simulink model "single_motor_fix"  (R2025b)
settings: Solver=VariableStepAuto  StartTime=0.0  StopTime=10.0  RelTol=1e-3
values from neighbouring files (symbols this model uses):
  Dm = 1e-3    (= 0.001)    [motor_param.m]
  Jm = 0.1e-3    (= 0.0001)    [motor_param.m]
  Ld = 0.01    [motor_param.m]
  Lq = 0.02    [motor_param.m]
  p = 2    [motor_param.m]
  Phi = 0.1    [motor_param.m]
  Rs = 0.38    [motor_param.m]
libraries: fl_lib x20, nesl_utility x20, ee_lib x6, eeTransforms x4, simulink x2
(part 1 of 2)
settings Model: Creator=ZhiyongXu  LastModifiedBy=ZhiyongXu

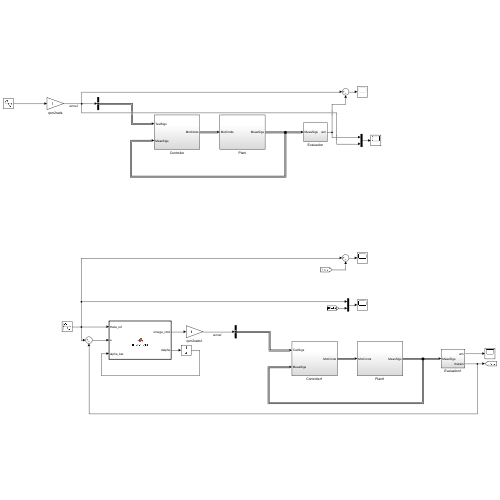
[thumbnail: Simulink's stored preview of the top-level diagram]
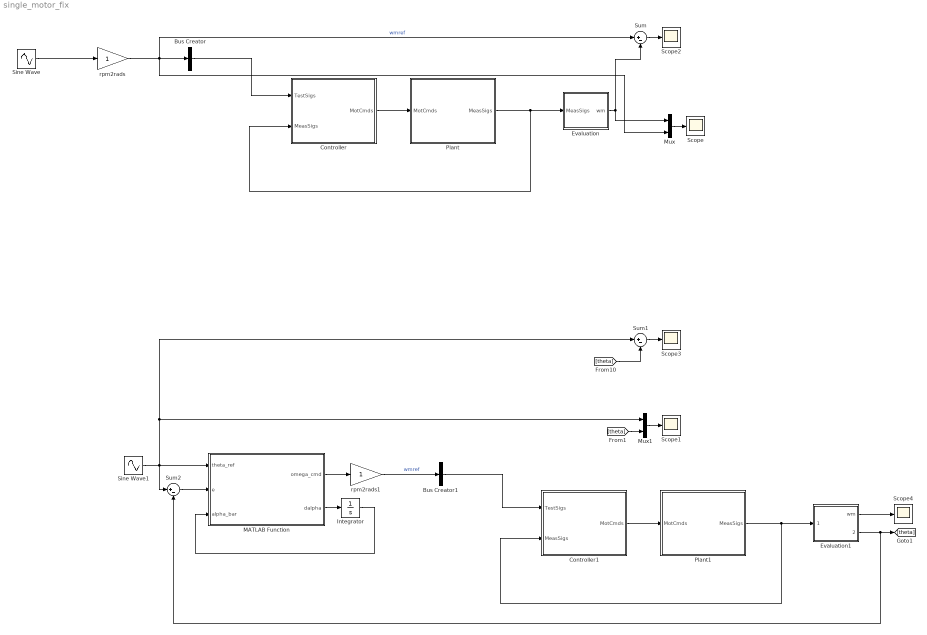
== system single_motor_fix ==
  Bus Creator : BusCreator  Inputs=1
  Bus Creator1 : BusCreator  Inputs=1
  Controller : Subsystem
  Controller1 : Subsystem
  Evaluation : Subsystem
  Evaluation1 : Subsystem
  Integrator : Integrator
  MATLAB Function : MATLAB Function  TreatAsAtomicUnit=on
  Mux : Mux  Inputs=2
  Mux1 : Mux  Inputs=2
  Plant : Subsystem
  Plant1 : Subsystem
  Scope{,1..4} (5 alike) : Scope
      Scope settings: ActiveDisplayYMinimum=-13.02025826891459  ActiveDisplayYMaximum=15.222741821849503
      Scope1 settings: ActiveDisplayYMinimum=-12.501085147532748  ActiveDisplayYMaximum=12.501085862817705  DataLoggingVariableName=ScopeData4
      Scope2 settings: ActiveDisplayYMinimum=-13.020433528439366  ActiveDisplayYMaximum=12.247347842337303  DataLoggingVariableName=ScopeData3
      Scope3 settings: ActiveDisplayYMinimum=-0.029985345068735  ActiveDisplayYMaximum=0.055166420482078135  DataLoggingVariableName=ScopeData5
      Scope4 settings: DataLoggingVariableName=ScopeData6
  Sine Wave : Sin  Amplitude=10  SampleTime=0
  Sine Wave1 : Sin  Amplitude=10  SampleTime=0
  Sum : Sum  Inputs=|+-
  Sum1 : Sum  Inputs=|+-
  Sum2 : Sum  Inputs=|+-
  rpm2rads : Gain
  rpm2rads1 : Gain
  wires:
  Controller/1(MotCmds) -> Plant/1(MotCmds)
  Sine Wave/1 -> rpm2rads/1
  Bus Creator/1 -> Controller/1(TestSigs)
  Plant/1(MeasSigs) -> Evaluation/1(MeasSigs), Controller/2(MeasSigs)
  rpm2rads/1 -> Sum/1, Mux/2, Bus Creator/1  "wmref"
  Mux/1 -> Scope/1
  Evaluation/1(wm) -> Mux/1, Sum/2
  Sum/1 -> Scope2/1
  MATLAB Function/2(dalpha) -> Integrator/1
  rpm2rads1/1 -> Bus Creator1/1  "wmref"
  Evaluation1/2(thetam) -> [theta], Sum2/2
  Evaluation1/1(wm) -> Scope4/1
  Mux1/1 -> Scope1/1
  [theta] -> Sum1/2
  Integrator/1 -> MATLAB Function/3(alpha_bar)
  MATLAB Function/1(omega_cmd) -> rpm2rads1/1
  Sum1/1 -> Scope3/1
  [theta] -> Mux1/2
  Sine Wave1/1 -> Mux1/1, Sum1/1, Sum2/1, MATLAB Function/1(theta_ref)
  Sum2/1 -> MATLAB Function/2(e)
  Bus Creator1/1 -> Controller1/1(TestSigs)
  Plant1/1(MeasSigs) -> Evaluation1/1(MeasSigs), Controller1/2(MeasSigs)
  Controller1/1(MotCmds) -> Plant1/1(MotCmds)

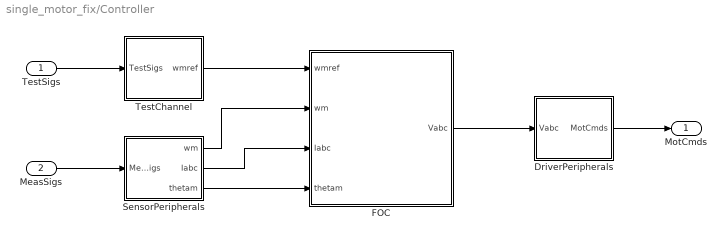
== system single_motor_fix/Controller ==
  TestSigs : Inport
  MeasSigs : Inport  Port=2
  DriverPeripherals : Subsystem
  FOC : Subsystem
  SensorPeripherals : Subsystem
  TestChannel : Subsystem
  MotCmds : Outport  VectorParamsAs1DForOutWhenUnconnected=off
  wires:
  FOC/1(Vabc) -> DriverPeripherals/1(Vabc)
  DriverPeripherals/1(MotCmds) -> MotCmds/1
  TestSigs/1 -> TestChannel/1(TestSigs)
  TestChannel/1(wmref) -> FOC/1(wmref)
  MeasSigs/1 -> SensorPeripherals/1(MeasSigs)
  SensorPeripherals/1(wm) -> FOC/2(wm)
  SensorPeripherals/2(Iabc) -> FOC/3(Iabc)
  SensorPeripherals/3(thetam) -> FOC/4(thetam)

== system single_motor_fix/Controller1 ==
  TestSigs : Inport
  MeasSigs : Inport  Port=2
  DriverPeripherals : Subsystem
  FOC : Subsystem
  SensorPeripherals : Subsystem
  TestChannel : Subsystem
  MotCmds : Outport  VectorParamsAs1DForOutWhenUnconnected=off
  wires:
  FOC/1(Vabc) -> DriverPeripherals/1(Vabc)
  DriverPeripherals/1(MotCmds) -> MotCmds/1
  TestSigs/1 -> TestChannel/1(TestSigs)
  TestChannel/1(wmref) -> FOC/1(wmref)
  MeasSigs/1 -> SensorPeripherals/1(MeasSigs)
  SensorPeripherals/1(wm) -> FOC/2(wm)
  SensorPeripherals/2(Iabc) -> FOC/3(Iabc)
  SensorPeripherals/3(thetam) -> FOC/4(thetam)

== system single_motor_fix/Evaluation ==
  MeasSigs : Inport
  Bus Selector1 : BusSelector  OutputSignals=wm,thetam
  Scope : Scope
      settings: ActiveDisplayYMinimum=-5.5392513465230095  ActiveDisplayYMaximum=26.372538555765981  DataLoggingVariableName=ScopeData2
  wm : Outport
  wires:
  MeasSigs/1 -> Bus Selector1/1
  Bus Selector1/2 -> Scope/1  "<thetam>"
  Bus Selector1/1 -> wm/1  "<wm>"

== system single_motor_fix/Evaluation1 ==
  MeasSigs : Inport
  Bus Selector1 : BusSelector  OutputSignals=wm,thetam
  wm : Outport
  thetam : Outport  Port=2
  wires:
  MeasSigs/1 -> Bus Selector1/1
  Bus Selector1/1 -> wm/1  "<wm>"
  Bus Selector1/2 -> thetam/1  "<thetam>"

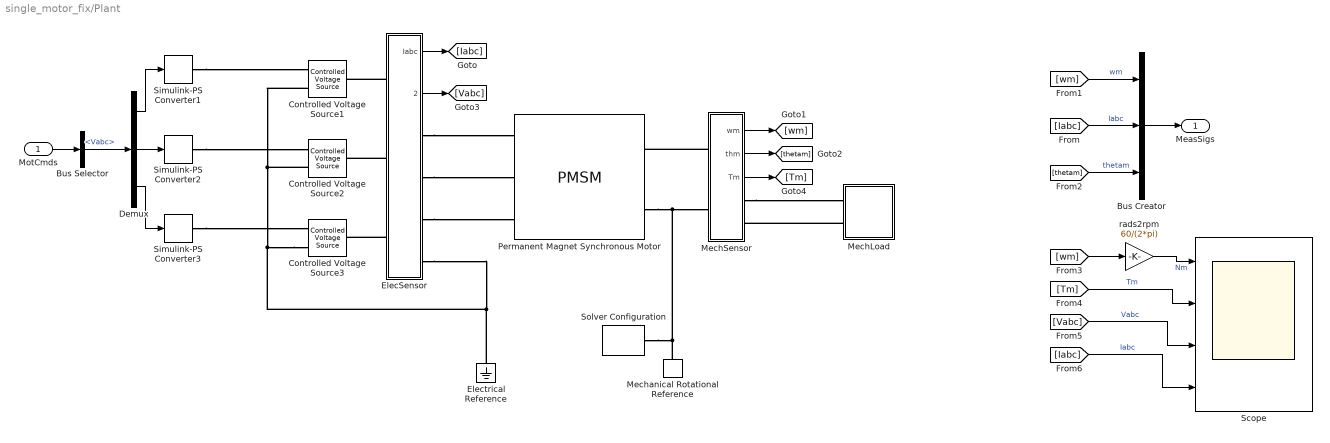
== system single_motor_fix/Plant ==
  MotCmds : Inport
  Bus Creator : BusCreator  Inputs=3
  Bus Selector : BusSelector  OutputSignals=Vabc
  Controlled Voltage Source1 : fl_lib/Electrical/Electrical Sources/Controlled Voltage Source
  Controlled Voltage Source2 : fl_lib/Electrical/Electrical Sources/Controlled Voltage Source
  Controlled Voltage Source3 : fl_lib/Electrical/Electrical Sources/Controlled Voltage Source
  Demux : Demux  Outputs=3
  ElecSensor : Subsystem
  Electrical Reference : fl_lib/Electrical/Electrical Elements/Electrical Reference
  MechLoad : Subsystem
  MechSensor : Subsystem
  Mechanical Rotational Reference : fl_lib/Mechanical/Rotational Elements/Mechanical Rotational Reference
  Permanent Magnet Synchronous Motor : ee_lib/Electromechanical/Permanent Magnet/PMSM  port_option=ee.enum.threePhasePort.expanded  winding_type=ee.enum.statorconnection.wye  machine_param=ee.enum.pmsm.parameterization.constant  nPolePairs=p  pmflux_param=1  pm_flux_linkage=Phi Wb  torque_constant=0.18 N*m/A  back_emf_constant=0.18 V/(rad/s)  stator_param=1  Ld=Ld H  Lq=Lq H  idVec=[-200, 0, 200] A  iqVec=[-200, 0, 200] A  LdMatrix=0.0002 * ones(3, 3) H  LqMatrix=0.0002 * ones(3, 3) H  PmMatrix=0.1 * ones(3, 3) Wb  ktMatrix=0.18 * ones(3, 3) N*m/A  keMatrix=0.18 * ones(3, 3) V/(rad/s)  L0=0 H  Ls=0.0002 H  Lm=-0.00002 H  Ms=0.00002 H  Rs=Rs Ohm  zero_sequence=ee.enum.park.zerosequence.exclude  axes_param=2  loss_param=ee.enum.ironloss.none  losses_oc=[0, 0, 0] W  losses_sc=[0, 0, 0] W  f_losses=60 Hz  Isc_losses=95 A  J=0 kg*m^2  lam=0 N*m/(rad/s)  i_d_specify=off  i_d_priority=None  i_d=0 A  i_d_nominal_specify=off  i_d_nominal_value=1  i_d_nominal_unit=A  i_q_specify=off  i_q_priority=None  i_q=0 A  i_q_nominal_specify=off  i_q_nominal_value=1  i_q_nominal_unit=A  torque_specify=off  torque_priority=None  torque=0 N*m  torque_nominal_specify=off  torque_nominal_value=1  torque_nominal_unit=N*m  angular_velocity_specify=on  angular_velocity_priority=High  angular_velocity=100 rpm  angular_velocity_nominal_specify=off  angular_velocity_nominal_value=1  angular_velocity_nominal_unit=rpm  angular_position_specify=off  angular_position_priority=High  angular_position=-2 rad  angular_position_nominal_specify=on  angular_position_nominal_value=100  angular_position_nominal_unit=deg  alpha=3.93e-3 1/K  alpha_flux=-0.001 1/K  Tmeas=298.15 K  stator_thermal_mass=100 J/K  rotor_thermal_mass=200 J/K  Rm_percent_rotor=90  Rd_percent_rotor=30  temperatureA_specify=off  temperatureA_priority=High  temperatureA=25 degC  temperatureA_nominal_specify=off  temperatureA_nominal_value=1  temperatureA_nominal_unit=degC  temperatureB_specify=off  temperatureB_priority=High  temperatureB=25 degC  temperatureB_nominal_specify=off  temperatureB_nominal_value=1  temperatureB_nominal_unit=degC  temperatureC_specify=off  temperatureC_priority=High  temperatureC=25 degC  temperatureC_nominal_specify=off  temperatureC_nominal_value=1  temperatureC_nominal_unit=degC  temperatureR_specify=off  temperatureR_priority=High  temperatureR=25 degC  temperatureR_nominal_specify=off  temperatureR_nominal_value=1  temperatureR_nominal_unit=degC
      settings: InternalSimscapePortConfiguration="{\"Bottom\":[],\"Left\":[{\"id\":\"a\",\"label\":\"a\",\"type\":\"foundation.electrical.electrical\"},{\"id\":\"b\",\"label\":\"b\",\"type\":\"foundation.electrical.electrical\"},{\"id\":\"c\",\"label\":\"c\",\"type\":\"foundation.electrical.electrical\"}],\"Right\":[{\"id\":\"R\",\"label\":\"R\",\"type\":\"foundation.mechanical.rotational.rotational\"},{\"id\":\"C\",\"label\":\"C\",\"type\":\"foundation.mechanical.rotational.rotational\"}],\"Top\":[]}"
  Scope : Scope  NumInputPorts=4
      settings: ActiveDisplayYMinimum=-41.571881527441555  ActiveDisplayYMaximum=115.73020905860461
  Simulink-PS Converter1 : nesl_utility/Simulink-PS Converter  PhysicalDomain=network_engine_domain  SubClassName=ps_input  LeftPortType=input  RightPortType=output  PseudoPeriodic=off  Frequencies=[]  NoiseDistribution=none  NoiseParameters=[]  Unit=1  AffineConversion=off  FilteringAndDerivatives=provide  SimscapeFilterOrder=1  InputFilterTimeConstant=1e-6  UdotUserProvided=0
  Simulink-PS Converter2 : nesl_utility/Simulink-PS Converter  PhysicalDomain=network_engine_domain  SubClassName=ps_input  LeftPortType=input  RightPortType=output  PseudoPeriodic=off  Frequencies=[]  NoiseDistribution=none  NoiseParameters=[]  Unit=1  AffineConversion=off  FilteringAndDerivatives=provide  SimscapeFilterOrder=1  InputFilterTimeConstant=1e-6  UdotUserProvided=0
  Simulink-PS Converter3 : nesl_utility/Simulink-PS Converter  PhysicalDomain=network_engine_domain  SubClassName=ps_input  LeftPortType=input  RightPortType=output  PseudoPeriodic=off  Frequencies=[]  NoiseDistribution=none  NoiseParameters=[]  Unit=1  AffineConversion=off  FilteringAndDerivatives=provide  SimscapeFilterOrder=1  InputFilterTimeConstant=1e-6  UdotUserProvided=0
  Solver Configuration : nesl_utility/Solver Configuration  PhysicalDomain=network_engine_domain  SubClassName=solver  LeftPortType=input  RightPortType=generic  Tones=[]  Harmonics=[]  SimulateNoise=off  Profile=off  UseLocalSampling=off  EnableSwitchedLinearOptims=on  FrequencyDomain=off  UseCCode=off  RelTol=0.001  AbsTol=1e-06  MinStep=1e-09  ToWorkspace=off  RevertToSquareIcSolve=off  NumHomotopyIterations=100  PhasorMode=off  PhasorModeNumHarmonics=1  ConsistencySolver=NEWTON_XTOL_AFTER_FTOL  IndexReductionMethod=DerivativeReplacement  DoDC=off  ResidualTolerance=1e-09  ConsistencyTolSource=GLOBAL  ConsistencyAbsTol=0.001  ConsistencyRelTol=0.001  ConsistencyTolFactor=0.001  UseLocalSolver=off  LocalSolverChoice=NE_BACKWARD_EULER_ADVANCER  ResolveIndetEquations=on  FunctionEvalNumThread=1  LocalSolverSampleTime=0.001  DoFixedCost=off  MaxNonlinIter=3  MaxModeIter=2  ComputeImpulses=off  ImpulseIterations=2  LinearAlgebra=Sparse  LinearAlgebraNumThread=0  EquationFormulation=NE_TIME_EF  DelaysMemoryBudget=1024  AutomaticFiltering=on  FilteringTimeConstant=0.001  PartitionStorageMethod=AS_NEEDED  PartitionMemoryBudget=1024  PartitionMethod=FAST  MultibodyUseLocalSolver=off  MultibodyLocalSolverChoice=ODE1  MultibodyLocalSolverSampleTime=0.001
  rads2rpm : Gain  Gain=60/(2*pi)
  MeasSigs : Outport  VectorParamsAs1DForOutWhenUnconnected=off
  wires:
  ElecSensor/1(Iabc) -> [Iabc]
  ElecSensor/2(Vabc) -> [Vabc]
  Demux/2 -> Simulink-PS Converter2/1
  Demux/1 -> Simulink-PS Converter1/1
  Demux/3 -> Simulink-PS Converter3/1
  MechSensor/1(wm) -> [wm]
  MechSensor/2(thm) -> [thetam]
  MechSensor/3(Tm) -> [Tm]
  [wm] -> Bus Creator/1  "wm"
  [Iabc] -> Bus Creator/2  "Iabc"
  [thetam] -> Bus Creator/3  "thetam"
  Bus Creator/1 -> MeasSigs/1
  MotCmds/1 -> Bus Selector/1
  Bus Selector/1 -> Demux/1  "<Vabc>"
  [wm] -> rads2rpm/1
  rads2rpm/1 -> Scope/1  "Nm"
  [Tm] -> Scope/2  "Tm"
  [Vabc] -> Scope/3  "Vabc"
  [Iabc] -> Scope/4  "Iabc"
  connections:
  Simulink-PS Converter2/RConn1 -- Controlled Voltage Source2/RConn1
  Simulink-PS Converter3/RConn1 -- Controlled Voltage Source3/RConn1
  ElecSensor/RConn3 -- Permanent Magnet Synchronous Motor/LConn3
  ElecSensor/LConn2 -- Controlled Voltage Source2/LConn1
  Controlled Voltage Source3/RConn2 -- Controlled Voltage Source1/RConn2 -- Controlled Voltage Source2/RConn2 -- ElecSensor/RConn4 -- Electrical Reference/LConn1
  ElecSensor/RConn2 -- Permanent Magnet Synchronous Motor/LConn2
  ElecSensor/RConn1 -- Permanent Magnet Synchronous Motor/LConn1
  ElecSensor/LConn3 -- Controlled Voltage Source3/LConn1
  ElecSensor/LConn1 -- Controlled Voltage Source1/LConn1
  Simulink-PS Converter1/RConn1 -- Controlled Voltage Source1/RConn1
  Permanent Magnet Synchronous Motor/RConn2 -- Solver Configuration/RConn1 -- Mechanical Rotational Reference/LConn1 -- MechSensor/LConn2
  MechSensor/RConn1 -- MechLoad/LConn1
  MechLoad/LConn2 -- MechSensor/RConn2
  MechSensor/LConn1 -- Permanent Magnet Synchronous Motor/RConn1

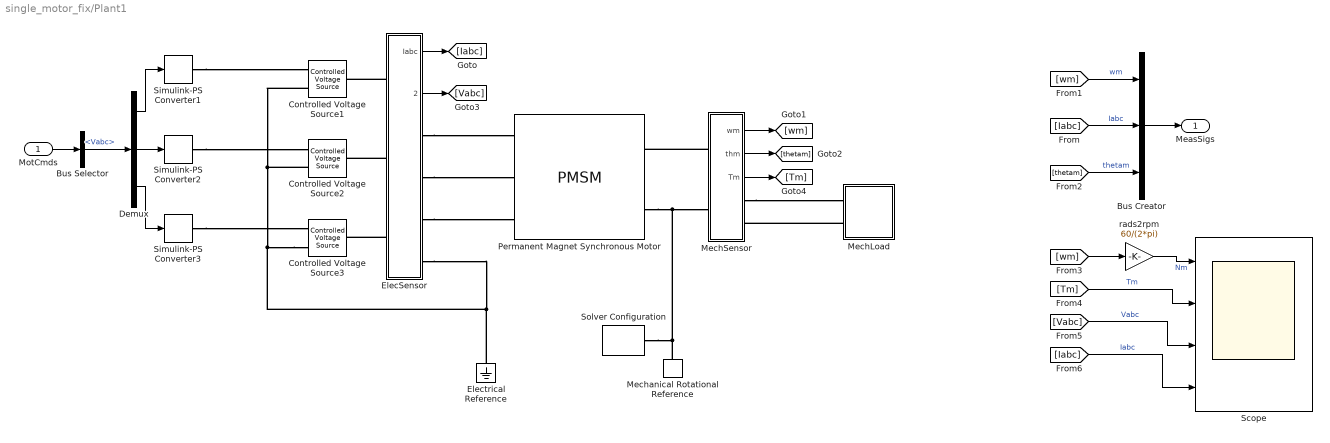
== system single_motor_fix/Plant1 ==
  MotCmds : Inport
  Bus Creator : BusCreator  Inputs=3
  Bus Selector : BusSelector  OutputSignals=Vabc
  Controlled Voltage Source1 : fl_lib/Electrical/Electrical Sources/Controlled Voltage Source
  Controlled Voltage Source2 : fl_lib/Electrical/Electrical Sources/Controlled Voltage Source
  Controlled Voltage Source3 : fl_lib/Electrical/Electrical Sources/Controlled Voltage Source
  Demux : Demux  Outputs=3
  ElecSensor : Subsystem
  Electrical Reference : fl_lib/Electrical/Electrical Elements/Electrical Reference
  MechLoad : Subsystem
  MechSensor : Subsystem
  Mechanical Rotational Reference : fl_lib/Mechanical/Rotational Elements/Mechanical Rotational Reference
  Permanent Magnet Synchronous Motor : ee_lib/Electromechanical/Permanent Magnet/PMSM  port_option=ee.enum.threePhasePort.expanded  winding_type=ee.enum.statorconnection.wye  machine_param=ee.enum.pmsm.parameterization.constant  nPolePairs=p  pmflux_param=1  pm_flux_linkage=Phi Wb  torque_constant=0.18 N*m/A  back_emf_constant=0.18 V/(rad/s)  stator_param=1  Ld=Ld H  Lq=Lq H  idVec=[-200, 0, 200] A  iqVec=[-200, 0, 200] A  LdMatrix=0.0002 * ones(3, 3) H  LqMatrix=0.0002 * ones(3, 3) H  PmMatrix=0.1 * ones(3, 3) Wb  ktMatrix=0.18 * ones(3, 3) N*m/A  keMatrix=0.18 * ones(3, 3) V/(rad/s)  L0=0 H  Ls=0.0002 H  Lm=-0.00002 H  Ms=0.00002 H  Rs=Rs Ohm  zero_sequence=ee.enum.park.zerosequence.exclude  axes_param=2  loss_param=ee.enum.ironloss.none  losses_oc=[0, 0, 0] W  losses_sc=[0, 0, 0] W  f_losses=60 Hz  Isc_losses=95 A  J=0 kg*m^2  lam=0 N*m/(rad/s)  i_d_specify=off  i_d_priority=None  i_d=0 A  i_d_nominal_specify=off  i_d_nominal_value=1  i_d_nominal_unit=A  i_q_specify=off  i_q_priority=None  i_q=0 A  i_q_nominal_specify=off  i_q_nominal_value=1  i_q_nominal_unit=A  torque_specify=off  torque_priority=None  torque=0 N*m  torque_nominal_specify=off  torque_nominal_value=1  torque_nominal_unit=N*m  angular_velocity_specify=on  angular_velocity_priority=High  angular_velocity=100 rpm  angular_velocity_nominal_specify=off  angular_velocity_nominal_value=1  angular_velocity_nominal_unit=rpm  angular_position_specify=off  angular_position_priority=High  angular_position=-2 rad  angular_position_nominal_specify=on  angular_position_nominal_value=100  angular_position_nominal_unit=deg  alpha=3.93e-3 1/K  alpha_flux=-0.001 1/K  Tmeas=298.15 K  stator_thermal_mass=100 J/K  rotor_thermal_mass=200 J/K  Rm_percent_rotor=90  Rd_percent_rotor=30  temperatureA_specify=off  temperatureA_priority=High  temperatureA=25 degC  temperatureA_nominal_specify=off  temperatureA_nominal_value=1  temperatureA_nominal_unit=degC  temperatureB_specify=off  temperatureB_priority=High  temperatureB=25 degC  temperatureB_nominal_specify=off  temperatureB_nominal_value=1  temperatureB_nominal_unit=degC  temperatureC_specify=off  temperatureC_priority=High  temperatureC=25 degC  temperatureC_nominal_specify=off  temperatureC_nominal_value=1  temperatureC_nominal_unit=degC  temperatureR_specify=off  temperatureR_priority=High  temperatureR=25 degC  temperatureR_nominal_specify=off  temperatureR_nominal_value=1  temperatureR_nominal_unit=degC
      settings: InternalSimscapePortConfiguration="{\"Bottom\":[],\"Left\":[{\"id\":\"a\",\"label\":\"a\",\"type\":\"foundation.electrical.electrical\"},{\"id\":\"b\",\"label\":\"b\",\"type\":\"foundation.electrical.electrical\"},{\"id\":\"c\",\"label\":\"c\",\"type\":\"foundation.electrical.electrical\"}],\"Right\":[{\"id\":\"R\",\"label\":\"R\",\"type\":\"foundation.mechanical.rotational.rotational\"},{\"id\":\"C\",\"label\":\"C\",\"type\":\"foundation.mechanical.rotational.rotational\"}],\"Top\":[]}"
  Scope : Scope  NumInputPorts=4
      settings: ActiveDisplayYMinimum=-41.571881527441555  ActiveDisplayYMaximum=115.73020905860461
  Simulink-PS Converter1 : nesl_utility/Simulink-PS Converter  PhysicalDomain=network_engine_domain  SubClassName=ps_input  LeftPortType=input  RightPortType=output  PseudoPeriodic=off  Frequencies=[]  NoiseDistribution=none  NoiseParameters=[]  Unit=1  AffineConversion=off  FilteringAndDerivatives=provide  SimscapeFilterOrder=1  InputFilterTimeConstant=1e-6  UdotUserProvided=0
  Simulink-PS Converter2 : nesl_utility/Simulink-PS Converter  PhysicalDomain=network_engine_domain  SubClassName=ps_input  LeftPortType=input  RightPortType=output  PseudoPeriodic=off  Frequencies=[]  NoiseDistribution=none  NoiseParameters=[]  Unit=1  AffineConversion=off  FilteringAndDerivatives=provide  SimscapeFilterOrder=1  InputFilterTimeConstant=1e-6  UdotUserProvided=0
  Simulink-PS Converter3 : nesl_utility/Simulink-PS Converter  PhysicalDomain=network_engine_domain  SubClassName=ps_input  LeftPortType=input  RightPortType=output  PseudoPeriodic=off  Frequencies=[]  NoiseDistribution=none  NoiseParameters=[]  Unit=1  AffineConversion=off  FilteringAndDerivatives=provide  SimscapeFilterOrder=1  InputFilterTimeConstant=1e-6  UdotUserProvided=0
  Solver Configuration : nesl_utility/Solver Configuration  PhysicalDomain=network_engine_domain  SubClassName=solver  LeftPortType=input  RightPortType=generic  Tones=[]  Harmonics=[]  SimulateNoise=off  Profile=off  UseLocalSampling=off  EnableSwitchedLinearOptims=on  FrequencyDomain=off  UseCCode=off  RelTol=0.001  AbsTol=1e-06  MinStep=1e-09  ToWorkspace=off  RevertToSquareIcSolve=off  NumHomotopyIterations=100  PhasorMode=off  PhasorModeNumHarmonics=1  ConsistencySolver=NEWTON_XTOL_AFTER_FTOL  IndexReductionMethod=DerivativeReplacement  DoDC=off  ResidualTolerance=1e-09  ConsistencyTolSource=GLOBAL  ConsistencyAbsTol=0.001  ConsistencyRelTol=0.001  ConsistencyTolFactor=0.001  UseLocalSolver=off  LocalSolverChoice=NE_BACKWARD_EULER_ADVANCER  ResolveIndetEquations=on  FunctionEvalNumThread=1  LocalSolverSampleTime=0.001  DoFixedCost=off  MaxNonlinIter=3  MaxModeIter=2  ComputeImpulses=off  ImpulseIterations=2  LinearAlgebra=Sparse  LinearAlgebraNumThread=0  EquationFormulation=NE_TIME_EF  DelaysMemoryBudget=1024  AutomaticFiltering=on  FilteringTimeConstant=0.001  PartitionStorageMethod=AS_NEEDED  PartitionMemoryBudget=1024  PartitionMethod=FAST  MultibodyUseLocalSolver=off  MultibodyLocalSolverChoice=ODE1  MultibodyLocalSolverSampleTime=0.001
  rads2rpm : Gain  Gain=60/(2*pi)
  MeasSigs : Outport  VectorParamsAs1DForOutWhenUnconnected=off
  wires:
  ElecSensor/1(Iabc) -> [Iabc]
  ElecSensor/2(Vabc) -> [Vabc]
  Demux/2 -> Simulink-PS Converter2/1
  Demux/1 -> Simulink-PS Converter1/1
  Demux/3 -> Simulink-PS Converter3/1
  MechSensor/1(wm) -> [wm]
  MechSensor/2(thm) -> [thetam]
  MechSensor/3(Tm) -> [Tm]
  [wm] -> Bus Creator/1  "wm"
  [Iabc] -> Bus Creator/2  "Iabc"
  [thetam] -> Bus Creator/3  "thetam"
  Bus Creator/1 -> MeasSigs/1
  MotCmds/1 -> Bus Selector/1
  Bus Selector/1 -> Demux/1  "<Vabc>"
  [wm] -> rads2rpm/1
  rads2rpm/1 -> Scope/1  "Nm"
  [Tm] -> Scope/2  "Tm"
  [Vabc] -> Scope/3  "Vabc"
  [Iabc] -> Scope/4  "Iabc"
  connections:
  Simulink-PS Converter2/RConn1 -- Controlled Voltage Source2/RConn1
  Simulink-PS Converter3/RConn1 -- Controlled Voltage Source3/RConn1
  ElecSensor/RConn3 -- Permanent Magnet Synchronous Motor/LConn3
  ElecSensor/LConn2 -- Controlled Voltage Source2/LConn1
  Controlled Voltage Source3/RConn2 -- Controlled Voltage Source1/RConn2 -- Controlled Voltage Source2/RConn2 -- ElecSensor/RConn4 -- Electrical Reference/LConn1
  ElecSensor/RConn2 -- Permanent Magnet Synchronous Motor/LConn2
  ElecSensor/RConn1 -- Permanent Magnet Synchronous Motor/LConn1
  ElecSensor/LConn3 -- Controlled Voltage Source3/LConn1
  ElecSensor/LConn1 -- Controlled Voltage Source1/LConn1
  Simulink-PS Converter1/RConn1 -- Controlled Voltage Source1/RConn1
  Permanent Magnet Synchronous Motor/RConn2 -- Solver Configuration/RConn1 -- Mechanical Rotational Reference/LConn1 -- MechSensor/LConn2
  MechSensor/RConn1 -- MechLoad/LConn1
  MechLoad/LConn2 -- MechSensor/RConn2
  MechSensor/LConn1 -- Permanent Magnet Synchronous Motor/RConn1

== system single_motor_fix/Controller/DriverPeripherals ==
  Vabc : Inport
  Break Algebraic Loop : Subsystem
  Bus Creator : BusCreator  Inputs=1
  MotCmds : Outport  VectorParamsAs1DForOutWhenUnconnected=off
  wires:
  Vabc/1 -> Break Algebraic Loop/1(In1)
  Bus Creator/1 -> MotCmds/1
  Break Algebraic Loop/1(Out1) -> Bus Creator/1  "Vabc"

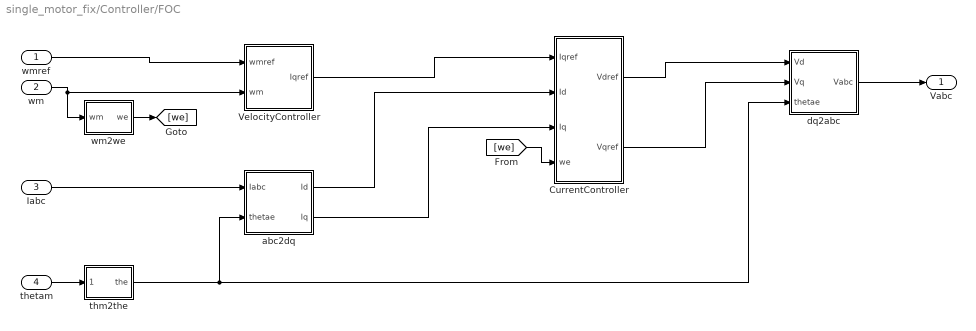
== system single_motor_fix/Controller/FOC ==
  wmref : Inport
  wm : Inport  Port=2
  Iabc : Inport  Port=3
  thetam : Inport  Port=4
  CurrentController : Subsystem
  VelocityController : Subsystem
  abc2dq : Subsystem
  dq2abc : Subsystem
  thm2the : Subsystem
  wm2we : Subsystem
  Vabc : Outport  VectorParamsAs1DForOutWhenUnconnected=off
  wires:
  abc2dq/2(Iq) -> CurrentController/3(Iq)
  wmref/1 -> VelocityController/1(wmref)
  abc2dq/1(Id) -> CurrentController/2(Id)
  Iabc/1 -> abc2dq/1(Iabc)
  CurrentController/1(Vdref) -> dq2abc/1(Vd)
  CurrentController/2(Vqref) -> dq2abc/2(Vq)
  [we] -> CurrentController/4(we)
  wm/1 -> VelocityController/2(wm), wm2we/1(wm)
  dq2abc/1(Vabc) -> Vabc/1
  VelocityController/1(Iqref) -> CurrentController/1(Iqref)
  thm2the/1(the) -> abc2dq/2(thetae), dq2abc/3(thetae)
  thetam/1 -> thm2the/1(thm)
  wm2we/1(we) -> [we]

== system single_motor_fix/Controller/SensorPeripherals ==
  MeasSigs : Inport
  Bus Selector : BusSelector  OutputSignals=wm,Iabc,thetam
  wm : Outport  VectorParamsAs1DForOutWhenUnconnected=off
  Iabc : Outport  Port=2  VectorParamsAs1DForOutWhenUnconnected=off
  thetam : Outport  Port=3  VectorParamsAs1DForOutWhenUnconnected=off
  wires:
  MeasSigs/1 -> Bus Selector/1
  Bus Selector/2 -> Iabc/1  "<Iabc>"
  Bus Selector/1 -> wm/1  "<wm>"
  Bus Selector/3 -> thetam/1  "<thetam>"

== system single_motor_fix/Controller/TestChannel ==
  TestSigs : Inport
  Bus Selector : BusSelector  OutputSignals=wmref
  wmref : Outport  VectorParamsAs1DForOutWhenUnconnected=off
  wires:
  TestSigs/1 -> Bus Selector/1
  Bus Selector/1 -> wmref/1  "<wmref>"

== system single_motor_fix/Controller1/DriverPeripherals ==
  Vabc : Inport
  Break Algebraic Loop : Subsystem
  Bus Creator : BusCreator  Inputs=1
  MotCmds : Outport  VectorParamsAs1DForOutWhenUnconnected=off
  wires:
  Vabc/1 -> Break Algebraic Loop/1(In1)
  Bus Creator/1 -> MotCmds/1
  Break Algebraic Loop/1(Out1) -> Bus Creator/1  "Vabc"

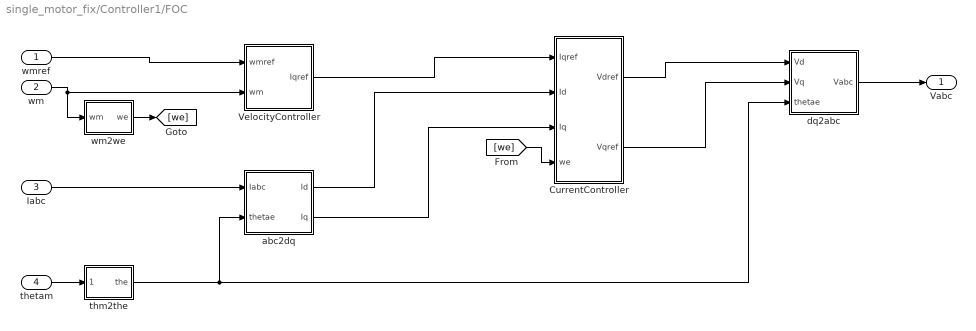
== system single_motor_fix/Controller1/FOC ==
  wmref : Inport
  wm : Inport  Port=2
  Iabc : Inport  Port=3
  thetam : Inport  Port=4
  CurrentController : Subsystem
  VelocityController : Subsystem
  abc2dq : Subsystem
  dq2abc : Subsystem
  thm2the : Subsystem
  wm2we : Subsystem
  Vabc : Outport  VectorParamsAs1DForOutWhenUnconnected=off
  wires:
  abc2dq/2(Iq) -> CurrentController/3(Iq)
  wmref/1 -> VelocityController/1(wmref)
  abc2dq/1(Id) -> CurrentController/2(Id)
  Iabc/1 -> abc2dq/1(Iabc)
  CurrentController/1(Vdref) -> dq2abc/1(Vd)
  CurrentController/2(Vqref) -> dq2abc/2(Vq)
  [we] -> CurrentController/4(we)
  wm/1 -> VelocityController/2(wm), wm2we/1(wm)
  dq2abc/1(Vabc) -> Vabc/1
  VelocityController/1(Iqref) -> CurrentController/1(Iqref)
  thm2the/1(the) -> abc2dq/2(thetae), dq2abc/3(thetae)
  thetam/1 -> thm2the/1(thm)
  wm2we/1(we) -> [we]

== system single_motor_fix/Controller1/SensorPeripherals ==
  MeasSigs : Inport
  Bus Selector : BusSelector  OutputSignals=wm,Iabc,thetam
  wm : Outport  VectorParamsAs1DForOutWhenUnconnected=off
  Iabc : Outport  Port=2  VectorParamsAs1DForOutWhenUnconnected=off
  thetam : Outport  Port=3  VectorParamsAs1DForOutWhenUnconnected=off
  wires:
  MeasSigs/1 -> Bus Selector/1
  Bus Selector/2 -> Iabc/1  "<Iabc>"
  Bus Selector/1 -> wm/1  "<wm>"
  Bus Selector/3 -> thetam/1  "<thetam>"

== system single_motor_fix/Controller1/TestChannel ==
  TestSigs : Inport
  Bus Selector : BusSelector  OutputSignals=wmref
  wmref : Outport  VectorParamsAs1DForOutWhenUnconnected=off
  wires:
  TestSigs/1 -> Bus Selector/1
  Bus Selector/1 -> wmref/1  "<wmref>"

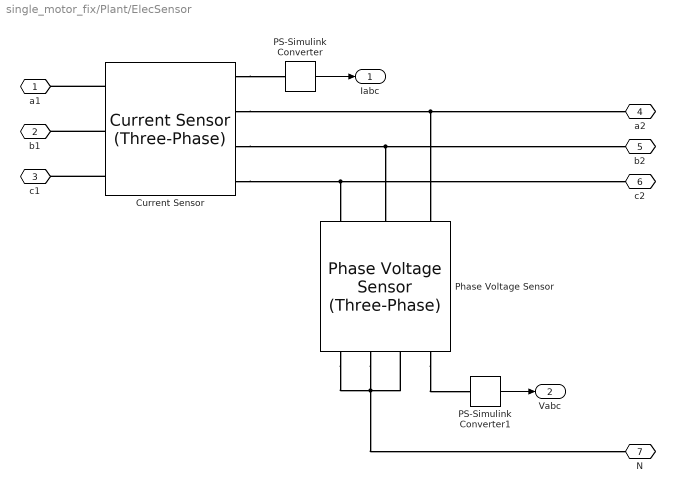
== system single_motor_fix/Plant/ElecSensor ==
  Current Sensor : ee_lib/Sensors & Transducers/Current Sensor (Three-Phase)
      settings: InternalSimscapePortConfiguration="{\"Bottom\":[],\"Left\":[{\"id\":\"a1\",\"label\":\"a1\",\"type\":\"foundation.electrical.electrical\"},{\"id\":\"b1\",\"label\":\"b1\",\"type\":\"foundation.electrical.electrical\"},{\"id\":\"c1\",\"label\":\"c1\",\"type\":\"foundation.electrical.electrical\"}],\"Right\":[{\"id\":\"I_output\",\"label\":\"I\",\"type\":\"output\"},{\"id\":\"a2\",\"label\":\"a2\",\"type\":\"foundation.electrical.electrical\"},{\"id\":\"b2\",\"label\":\"b2\",\"type\":\"foundation.electrical.electrical\"},{\"id\":\"c2\",\"label\":\"c2\",\"type\":\"foundation.electrical.electrical\"}],\"Top\":[]}"
  PS-Simulink Converter : nesl_utility/PS-Simulink Converter  PhysicalDomain=network_engine_domain  SubClassName=ps_output  LeftPortType=input  RightPortType=output  PseudoPeriodic=off  Frequencies=[]  VectorFormat=1-D array  Unit=1  AffineConversion=off
  PS-Simulink Converter1 : nesl_utility/PS-Simulink Converter  PhysicalDomain=network_engine_domain  SubClassName=ps_output  LeftPortType=input  RightPortType=output  PseudoPeriodic=off  Frequencies=[]  VectorFormat=1-D array  Unit=1  AffineConversion=off
  Phase Voltage Sensor : ee_lib/Sensors & Transducers/Phase Voltage Sensor (Three-Phase)
      settings: InternalSimscapePortConfiguration="{\"Bottom\":[],\"Left\":[{\"id\":\"a1\",\"label\":\"a1\",\"type\":\"foundation.electrical.electrical\"},{\"id\":\"b1\",\"label\":\"b1\",\"type\":\"foundation.electrical.electrical\"},{\"id\":\"c1\",\"label\":\"c1\",\"type\":\"foundation.electrical.electrical\"}],\"Right\":[{\"id\":\"V_output\",\"label\":\"V\",\"type\":\"output\"},{\"id\":\"a2\",\"label\":\"a2\",\"type\":\"foundation.electrical.electrical\"},{\"id\":\"b2\",\"label\":\"b2\",\"type\":\"foundation.electrical.electrical\"},{\"id\":\"c2\",\"label\":\"c2\",\"type\":\"foundation.electrical.electrical\"}],\"Top\":[]}"
  a1 : PMIOPort  Side=Left
  b1 : PMIOPort  Port=2  Side=Left
  c1 : PMIOPort  Port=3  Side=Left
  a2 : PMIOPort  Port=4  Side=Right
  b2 : PMIOPort  Port=5  Side=Right
  c2 : PMIOPort  Port=6  Side=Right
  N : PMIOPort  Port=7  Side=Right
  Iabc : Outport  VectorParamsAs1DForOutWhenUnconnected=off
  Vabc : Outport  Port=2  VectorParamsAs1DForOutWhenUnconnected=off
  wires:
  PS-Simulink Converter/1 -> Iabc/1
  PS-Simulink Converter1/1 -> Vabc/1
  connections:
  Current Sensor/LConn1 -- a1/RConn1
  Current Sensor/LConn2 -- b1/RConn1
  Current Sensor/LConn3 -- c1/RConn1
  Current Sensor/RConn1 -- PS-Simulink Converter/LConn1
  Phase Voltage Sensor/RConn1 -- PS-Simulink Converter1/LConn1
  Current Sensor/RConn2 -- a2/RConn1 -- Phase Voltage Sensor/LConn1
  Current Sensor/RConn3 -- b2/RConn1 -- Phase Voltage Sensor/LConn2
  Current Sensor/RConn4 -- c2/RConn1 -- Phase Voltage Sensor/LConn3
  Phase Voltage Sensor/RConn4 -- N/RConn1 -- Phase Voltage Sensor/RConn3 -- Phase Voltage Sensor/RConn2

== system single_motor_fix/Plant/MechLoad ==
  Ideal Torque Source : fl_lib/Mechanical/Mechanical Sources/Ideal Torque Source
  Inertia : fl_lib/Mechanical/Rotational Elements/Inertia  inertia=Jm kg*m^2  num_ports=foundation.enum.numPorts2.one  w_specify=on  w_priority=High  w=100 rpm  w_nominal_specify=off  w_nominal_value=1  w_nominal_unit=rad/s  t_specify=off  t_priority=None  t=0 N*m  t_nominal_specify=off  t_nominal_value=1  t_nominal_unit=N*m
  Repeating Sequence : simulink/Sources/Repeating Sequence  rep_seq_t=[0 5]  rep_seq_y=[0 2]
  Rotational Damper : fl_lib/Mechanical/Rotational Elements/Rotational Damper  D=Dm N*m/(rad/s)  w_specify=off  w_priority=None  w=0 rad/s  w_nominal_specify=off  w_nominal_value=1  w_nominal_unit=rad/s  t_specify=off  t_priority=None  t=0 N*m  t_nominal_specify=off  t_nominal_value=1  t_nominal_unit=N*m
  Simulink-PS Converter4 : nesl_utility/Simulink-PS Converter  PhysicalDomain=network_engine_domain  SubClassName=ps_input  LeftPortType=input  RightPortType=output  PseudoPeriodic=off  Frequencies=[]  NoiseDistribution=none  NoiseParameters=[]  Unit=1  AffineConversion=off  FilteringAndDerivatives=provide  SimscapeFilterOrder=1  InputFilterTimeConstant=0.001  UdotUserProvided=0
  R : PMIOPort  Side=Left
  C : PMIOPort  Port=2  Side=Left
  wires:
  Repeating Sequence/1 -> Simulink-PS Converter4/1
  connections:
  Ideal Torque Source/RConn1 -- Simulink-PS Converter4/RConn1
  Rotational Damper/RConn1 -- Ideal Torque Source/RConn2 -- C/RConn1
  Rotational Damper/LConn1 -- Ideal Torque Source/LConn1 -- R/RConn1 -- Inertia/LConn1

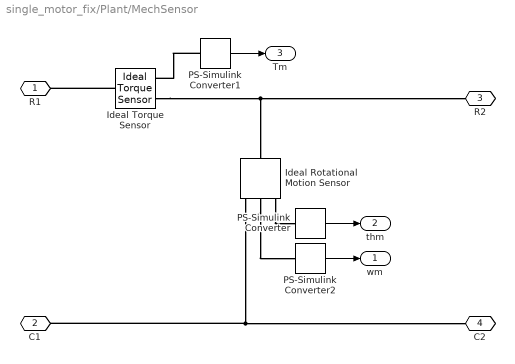
== system single_motor_fix/Plant/MechSensor ==
  Ideal Rotational Motion Sensor : fl_lib/Mechanical/Mechanical Sensors/Ideal Rotational Motion Sensor  reference=foundation.enum.MeasurementReference.difference  acceleration_port=false  velocity_port=true  position_port=true  wrap_angle=simscape.enum.onoff.off  offset=0 rad
  Ideal Torque Sensor : fl_lib/Mechanical/Mechanical Sensors/Ideal Torque Sensor
  PS-Simulink Converter : nesl_utility/PS-Simulink Converter  PhysicalDomain=network_engine_domain  SubClassName=ps_output  LeftPortType=input  RightPortType=output  PseudoPeriodic=off  Frequencies=[]  VectorFormat=1-D array  Unit=1  AffineConversion=off
  PS-Simulink Converter1 : nesl_utility/PS-Simulink Converter  PhysicalDomain=network_engine_domain  SubClassName=ps_output  LeftPortType=input  RightPortType=output  PseudoPeriodic=off  Frequencies=[]  VectorFormat=1-D array  Unit=1  AffineConversion=off
  PS-Simulink Converter2 : nesl_utility/PS-Simulink Converter  PhysicalDomain=network_engine_domain  SubClassName=ps_output  LeftPortType=input  RightPortType=output  PseudoPeriodic=off  Frequencies=[]  VectorFormat=1-D array  Unit=1  AffineConversion=off
  R1 : PMIOPort  Side=Left
  C1 : PMIOPort  Port=2  Side=Left
  R2 : PMIOPort  Port=3  Side=Right
  C2 : PMIOPort  Port=4  Side=Right
  wm : Outport  VectorParamsAs1DForOutWhenUnconnected=off
  thm : Outport  Port=2  VectorParamsAs1DForOutWhenUnconnected=off
  Tm : Outport  Port=3  VectorParamsAs1DForOutWhenUnconnected=off
  wires:
  PS-Simulink Converter/1 -> thm/1
  PS-Simulink Converter1/1 -> Tm/1
  PS-Simulink Converter2/1 -> wm/1
  connections:
  Ideal Rotational Motion Sensor/RConn3 -- PS-Simulink Converter/LConn1
  Ideal Rotational Motion Sensor/RConn1 -- C2/RConn1 -- C1/RConn1
  Ideal Torque Sensor/LConn1 -- R1/RConn1
  Ideal Torque Sensor/RConn1 -- R2/RConn1 -- Ideal Rotational Motion Sensor/LConn1
  PS-Simulink Converter1/LConn1 -- Ideal Torque Sensor/RConn2
  Ideal Rotational Motion Sensor/RConn2 -- PS-Simulink Converter2/LConn1

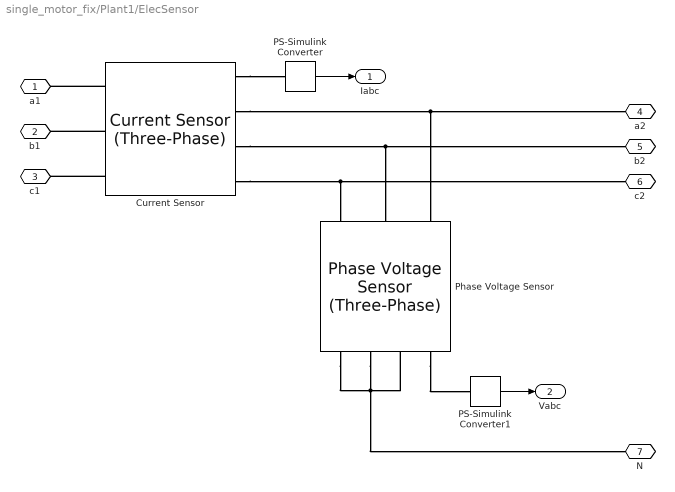
== system single_motor_fix/Plant1/ElecSensor ==
  Current Sensor : ee_lib/Sensors & Transducers/Current Sensor (Three-Phase)
      settings: InternalSimscapePortConfiguration="{\"Bottom\":[],\"Left\":[{\"id\":\"a1\",\"label\":\"a1\",\"type\":\"foundation.electrical.electrical\"},{\"id\":\"b1\",\"label\":\"b1\",\"type\":\"foundation.electrical.electrical\"},{\"id\":\"c1\",\"label\":\"c1\",\"type\":\"foundation.electrical.electrical\"}],\"Right\":[{\"id\":\"I_output\",\"label\":\"I\",\"type\":\"output\"},{\"id\":\"a2\",\"label\":\"a2\",\"type\":\"foundation.electrical.electrical\"},{\"id\":\"b2\",\"label\":\"b2\",\"type\":\"foundation.electrical.electrical\"},{\"id\":\"c2\",\"label\":\"c2\",\"type\":\"foundation.electrical.electrical\"}],\"Top\":[]}"
  PS-Simulink Converter : nesl_utility/PS-Simulink Converter  PhysicalDomain=network_engine_domain  SubClassName=ps_output  LeftPortType=input  RightPortType=output  PseudoPeriodic=off  Frequencies=[]  VectorFormat=1-D array  Unit=1  AffineConversion=off
  PS-Simulink Converter1 : nesl_utility/PS-Simulink Converter  PhysicalDomain=network_engine_domain  SubClassName=ps_output  LeftPortType=input  RightPortType=output  PseudoPeriodic=off  Frequencies=[]  VectorFormat=1-D array  Unit=1  AffineConversion=off
  Phase Voltage Sensor : ee_lib/Sensors & Transducers/Phase Voltage Sensor (Three-Phase)
      settings: InternalSimscapePortConfiguration="{\"Bottom\":[],\"Left\":[{\"id\":\"a1\",\"label\":\"a1\",\"type\":\"foundation.electrical.electrical\"},{\"id\":\"b1\",\"label\":\"b1\",\"type\":\"foundation.electrical.electrical\"},{\"id\":\"c1\",\"label\":\"c1\",\"type\":\"foundation.electrical.electrical\"}],\"Right\":[{\"id\":\"V_output\",\"label\":\"V\",\"type\":\"output\"},{\"id\":\"a2\",\"label\":\"a2\",\"type\":\"foundation.electrical.electrical\"},{\"id\":\"b2\",\"label\":\"b2\",\"type\":\"foundation.electrical.electrical\"},{\"id\":\"c2\",\"label\":\"c2\",\"type\":\"foundation.electrical.electrical\"}],\"Top\":[]}"
  a1 : PMIOPort  Side=Left
  b1 : PMIOPort  Port=2  Side=Left
  c1 : PMIOPort  Port=3  Side=Left
  a2 : PMIOPort  Port=4  Side=Right
  b2 : PMIOPort  Port=5  Side=Right
  c2 : PMIOPort  Port=6  Side=Right
  N : PMIOPort  Port=7  Side=Right
  Iabc : Outport  VectorParamsAs1DForOutWhenUnconnected=off
  Vabc : Outport  Port=2  VectorParamsAs1DForOutWhenUnconnected=off
  wires:
  PS-Simulink Converter/1 -> Iabc/1
  PS-Simulink Converter1/1 -> Vabc/1
  connections:
  Current Sensor/LConn1 -- a1/RConn1
  Current Sensor/LConn2 -- b1/RConn1
  Current Sensor/LConn3 -- c1/RConn1
  Current Sensor/RConn1 -- PS-Simulink Converter/LConn1
  Phase Voltage Sensor/RConn1 -- PS-Simulink Converter1/LConn1
  Current Sensor/RConn2 -- a2/RConn1 -- Phase Voltage Sensor/LConn1
  Current Sensor/RConn3 -- b2/RConn1 -- Phase Voltage Sensor/LConn2
  Current Sensor/RConn4 -- c2/RConn1 -- Phase Voltage Sensor/LConn3
  Phase Voltage Sensor/RConn4 -- N/RConn1 -- Phase Voltage Sensor/RConn3 -- Phase Voltage Sensor/RConn2

== system single_motor_fix/Plant1/MechLoad ==
  Ideal Torque Source : fl_lib/Mechanical/Mechanical Sources/Ideal Torque Source
  Inertia : fl_lib/Mechanical/Rotational Elements/Inertia  inertia=Jm kg*m^2  num_ports=foundation.enum.numPorts2.one  w_specify=on  w_priority=High  w=100 rpm  w_nominal_specify=off  w_nominal_value=1  w_nominal_unit=rad/s  t_specify=off  t_priority=None  t=0 N*m  t_nominal_specify=off  t_nominal_value=1  t_nominal_unit=N*m
  Repeating Sequence : simulink/Sources/Repeating Sequence  rep_seq_t=[0 5]  rep_seq_y=[0 2]
  Rotational Damper : fl_lib/Mechanical/Rotational Elements/Rotational Damper  D=Dm N*m/(rad/s)  w_specify=off  w_priority=None  w=0 rad/s  w_nominal_specify=off  w_nominal_value=1  w_nominal_unit=rad/s  t_specify=off  t_priority=None  t=0 N*m  t_nominal_specify=off  t_nominal_value=1  t_nominal_unit=N*m
  Simulink-PS Converter4 : nesl_utility/Simulink-PS Converter  PhysicalDomain=network_engine_domain  SubClassName=ps_input  LeftPortType=input  RightPortType=output  PseudoPeriodic=off  Frequencies=[]  NoiseDistribution=none  NoiseParameters=[]  Unit=1  AffineConversion=off  FilteringAndDerivatives=provide  SimscapeFilterOrder=1  InputFilterTimeConstant=0.001  UdotUserProvided=0
  R : PMIOPort  Side=Left
  C : PMIOPort  Port=2  Side=Left
  wires:
  Repeating Sequence/1 -> Simulink-PS Converter4/1
  connections:
  Ideal Torque Source/RConn1 -- Simulink-PS Converter4/RConn1
  Rotational Damper/RConn1 -- Ideal Torque Source/RConn2 -- C/RConn1
  Rotational Damper/LConn1 -- Ideal Torque Source/LConn1 -- R/RConn1 -- Inertia/LConn1

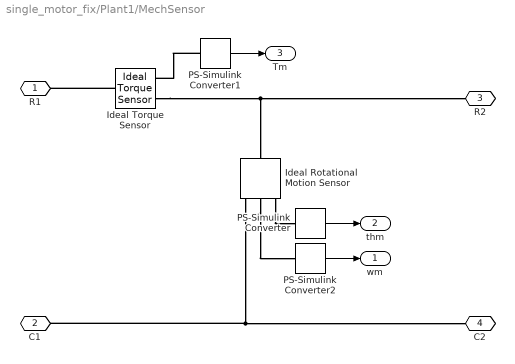
== system single_motor_fix/Plant1/MechSensor ==
  Ideal Rotational Motion Sensor : fl_lib/Mechanical/Mechanical Sensors/Ideal Rotational Motion Sensor  reference=foundation.enum.MeasurementReference.difference  acceleration_port=false  velocity_port=true  position_port=true  wrap_angle=simscape.enum.onoff.off  offset=0 rad
  Ideal Torque Sensor : fl_lib/Mechanical/Mechanical Sensors/Ideal Torque Sensor
  PS-Simulink Converter : nesl_utility/PS-Simulink Converter  PhysicalDomain=network_engine_domain  SubClassName=ps_output  LeftPortType=input  RightPortType=output  PseudoPeriodic=off  Frequencies=[]  VectorFormat=1-D array  Unit=1  AffineConversion=off
  PS-Simulink Converter1 : nesl_utility/PS-Simulink Converter  PhysicalDomain=network_engine_domain  SubClassName=ps_output  LeftPortType=input  RightPortType=output  PseudoPeriodic=off  Frequencies=[]  VectorFormat=1-D array  Unit=1  AffineConversion=off
  PS-Simulink Converter2 : nesl_utility/PS-Simulink Converter  PhysicalDomain=network_engine_domain  SubClassName=ps_output  LeftPortType=input  RightPortType=output  PseudoPeriodic=off  Frequencies=[]  VectorFormat=1-D array  Unit=1  AffineConversion=off
  R1 : PMIOPort  Side=Left
  C1 : PMIOPort  Port=2  Side=Left
  R2 : PMIOPort  Port=3  Side=Right
  C2 : PMIOPort  Port=4  Side=Right
  wm : Outport  VectorParamsAs1DForOutWhenUnconnected=off
  thm : Outport  Port=2  VectorParamsAs1DForOutWhenUnconnected=off
  Tm : Outport  Port=3  VectorParamsAs1DForOutWhenUnconnected=off
  wires:
  PS-Simulink Converter/1 -> thm/1
  PS-Simulink Converter1/1 -> Tm/1
  PS-Simulink Converter2/1 -> wm/1
  connections:
  Ideal Rotational Motion Sensor/RConn3 -- PS-Simulink Converter/LConn1
  Ideal Rotational Motion Sensor/RConn1 -- C2/RConn1 -- C1/RConn1
  Ideal Torque Sensor/LConn1 -- R1/RConn1
  Ideal Torque Sensor/RConn1 -- R2/RConn1 -- Ideal Rotational Motion Sensor/LConn1
  PS-Simulink Converter1/LConn1 -- Ideal Torque Sensor/RConn2
  Ideal Rotational Motion Sensor/RConn2 -- PS-Simulink Converter2/LConn1

== system single_motor_fix/Controller/DriverPeripherals/Break Algebraic Loop ==
  In1 : Inport
  Demux : Demux  Outputs=3
  Mux : Mux  Inputs=3
  Transfer Fcn : TransferFcn  Denominator=[1e-6 1]
  Transfer Fcn1 : TransferFcn  Denominator=[1e-6 1]
  Transfer Fcn2 : TransferFcn  Denominator=[1e-6 1]
  Out1 : Outport
  wires:
  In1/1 -> Demux/1
  Demux/1 -> Transfer Fcn/1
  Transfer Fcn/1 -> Mux/1
  Demux/2 -> Transfer Fcn1/1
  Transfer Fcn1/1 -> Mux/2
  Demux/3 -> Transfer Fcn2/1
  Transfer Fcn2/1 -> Mux/3
  Mux/1 -> Out1/1

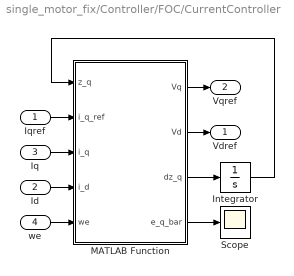
== system single_motor_fix/Controller/FOC/CurrentController ==
  Iqref : Inport
  Id : Inport  Port=2
  Iq : Inport  Port=3
  we : Inport  Port=4
  Integrator : Integrator
  MATLAB Function : MATLAB Function  TreatAsAtomicUnit=on
  Scope : Scope
      settings: ActiveDisplayYMinimum=-0.021972241997855933  ActiveDisplayYMaximum=0.011100987286103392  DataLoggingVariableName=ScopeData15
  Vdref : Outport  VectorParamsAs1DForOutWhenUnconnected=off
  Vqref : Outport  Port=2  VectorParamsAs1DForOutWhenUnconnected=off
  wires:
  MATLAB Function/2(Vd) -> Vdref/1
  Iqref/1 -> MATLAB Function/2(i_q_ref)
  MATLAB Function/4(e_q_bar) -> Scope/1
  we/1 -> MATLAB Function/5(we)
  Id/1 -> MATLAB Function/4(i_d)
  Iq/1 -> MATLAB Function/3(i_q)
  Integrator/1 -> MATLAB Function/1(z_q)
  MATLAB Function/1(Vq) -> Vqref/1
  MATLAB Function/3(dz_q) -> Integrator/1

== system single_motor_fix/Controller/FOC/VelocityController ==
  wmref : Inport
  wm : Inport  Port=2
  Gain : Gain  Gain=1/(3/2*p*Phi)
  Integrator : Integrator
  Integrator1 : Integrator
  MATLAB Function : MATLAB Function  TreatAsAtomicUnit=on
  Iqref : Outport  VectorParamsAs1DForOutWhenUnconnected=off
  wires:
  MATLAB Function/2(dot_bar_w) -> Integrator/1
  wm/1 -> MATLAB Function/2(w_m)
  MATLAB Function/1(u_cmd) -> Gain/1
  Integrator/1 -> MATLAB Function/3(bar_w)
  Gain/1 -> Iqref/1
  wmref/1 -> MATLAB Function/1(w_ref)
  MATLAB Function/3(dot_xi) -> Integrator1/1
  Integrator1/1 -> MATLAB Function/4(xi)

== system single_motor_fix/Controller/FOC/abc2dq ==
  Iabc : Inport
  thetae : Inport  Port=2
  Demux1 : Demux  Outputs=3
  Park Transform : eeTransforms/Park Transform  AxisAlignment=D-axis  PowerInvariant=off
  Terminator : Terminator
  Id : Outport  VectorParamsAs1DForOutWhenUnconnected=off
  Iq : Outport  Port=2  VectorParamsAs1DForOutWhenUnconnected=off
  wires:
  Iabc/1 -> Park Transform/1
  thetae/1 -> Park Transform/2
  Demux1/3 -> Terminator/1
  Park Transform/1 -> Demux1/1
  Demux1/1 -> Id/1
  Demux1/2 -> Iq/1

== system single_motor_fix/Controller/FOC/dq2abc ==
  Vd : Inport
  Vq : Inport  Port=2
  thetae : Inport  Port=3
  Constant : Constant  Value=0
  Inverse Park Transform : eeTransforms/Inverse Park Transform  AxisAlignment=D-axis  PowerInvariant=off
  Mux : Mux  Inputs=3
  Vabc : Outport  VectorParamsAs1DForOutWhenUnconnected=off
  wires:
  thetae/1 -> Inverse Park Transform/2
  Constant/1 -> Mux/3
  Mux/1 -> Inverse Park Transform/1
  Vd/1 -> Mux/1
  Inverse Park Transform/1 -> Vabc/1
  Vq/1 -> Mux/2

== system single_motor_fix/Controller/FOC/thm2the ==
  thm : Inport
  Constant : Constant  Value=2*pi
  Mod : Math  Operator=mod  SignedPower=on
  PolePairs : Gain  Gain=p
  the : Outport  VectorParamsAs1DForOutWhenUnconnected=off
  wires:
  Constant/1 -> Mod/2
  PolePairs/1 -> Mod/1
  Mod/1 -> the/1
  thm/1 -> PolePairs/1

== system single_motor_fix/Controller/FOC/wm2we ==
  wm : Inport
  PolePairs : Gain  Gain=p
  we : Outport  VectorParamsAs1DForOutWhenUnconnected=off
  wires:
  wm/1 -> PolePairs/1
  PolePairs/1 -> we/1

== system single_motor_fix/Controller1/DriverPeripherals/Break Algebraic Loop ==
  In1 : Inport
  Demux : Demux  Outputs=3
  Mux : Mux  Inputs=3
  Transfer Fcn : TransferFcn  Denominator=[1e-6 1]
  Transfer Fcn1 : TransferFcn  Denominator=[1e-6 1]
  Transfer Fcn2 : TransferFcn  Denominator=[1e-6 1]
  Out1 : Outport
  wires:
  In1/1 -> Demux/1
  Demux/1 -> Transfer Fcn/1
  Transfer Fcn/1 -> Mux/1
  Demux/2 -> Transfer Fcn1/1
  Transfer Fcn1/1 -> Mux/2
  Demux/3 -> Transfer Fcn2/1
  Transfer Fcn2/1 -> Mux/3
  Mux/1 -> Out1/1

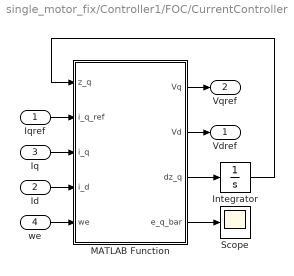
== system single_motor_fix/Controller1/FOC/CurrentController ==
  Iqref : Inport
  Id : Inport  Port=2
  Iq : Inport  Port=3
  we : Inport  Port=4
  Integrator : Integrator
  MATLAB Function : MATLAB Function  TreatAsAtomicUnit=on
  Scope : Scope
      settings: ActiveDisplayYMinimum=-0.021972241997855933  ActiveDisplayYMaximum=0.011100987286103392  DataLoggingVariableName=ScopeData15
  Vdref : Outport  VectorParamsAs1DForOutWhenUnconnected=off
  Vqref : Outport  Port=2  VectorParamsAs1DForOutWhenUnconnected=off
  wires:
  MATLAB Function/2(Vd) -> Vdref/1
  Iqref/1 -> MATLAB Function/2(i_q_ref)
  MATLAB Function/4(e_q_bar) -> Scope/1
  we/1 -> MATLAB Function/5(we)
  Id/1 -> MATLAB Function/4(i_d)
  Iq/1 -> MATLAB Function/3(i_q)
  Integrator/1 -> MATLAB Function/1(z_q)
  MATLAB Function/1(Vq) -> Vqref/1
  MATLAB Function/3(dz_q) -> Integrator/1

== system single_motor_fix/Controller1/FOC/VelocityController ==
  wmref : Inport
  wm : Inport  Port=2
  Gain : Gain  Gain=1/(3/2*p*Phi)
  Integrator : Integrator
  Integrator1 : Integrator
  MATLAB Function : MATLAB Function  TreatAsAtomicUnit=on
  Iqref : Outport  VectorParamsAs1DForOutWhenUnconnected=off
  wires:
  MATLAB Function/2(dot_bar_w) -> Integrator/1
  wm/1 -> MATLAB Function/2(w_m)
  MATLAB Function/1(u_cmd) -> Gain/1
  Integrator/1 -> MATLAB Function/3(bar_w)
  Gain/1 -> Iqref/1
  wmref/1 -> MATLAB Function/1(w_ref)
  MATLAB Function/3(dot_xi) -> Integrator1/1
  Integrator1/1 -> MATLAB Function/4(xi)

== system single_motor_fix/Controller1/FOC/abc2dq ==
  Iabc : Inport
  thetae : Inport  Port=2
  Demux1 : Demux  Outputs=3
  Park Transform : eeTransforms/Park Transform  AxisAlignment=D-axis  PowerInvariant=off
  Terminator : Terminator
  Id : Outport  VectorParamsAs1DForOutWhenUnconnected=off
  Iq : Outport  Port=2  VectorParamsAs1DForOutWhenUnconnected=off
  wires:
  Iabc/1 -> Park Transform/1
  thetae/1 -> Park Transform/2
  Demux1/3 -> Terminator/1
  Park Transform/1 -> Demux1/1
  Demux1/1 -> Id/1
  Demux1/2 -> Iq/1

== system single_motor_fix/Controller1/FOC/dq2abc ==
  Vd : Inport
  Vq : Inport  Port=2
  thetae : Inport  Port=3
  Constant : Constant  Value=0
  Inverse Park Transform : eeTransforms/Inverse Park Transform  AxisAlignment=D-axis  PowerInvariant=off
  Mux : Mux  Inputs=3
  Vabc : Outport  VectorParamsAs1DForOutWhenUnconnected=off
  wires:
  thetae/1 -> Inverse Park Transform/2
  Constant/1 -> Mux/3
  Mux/1 -> Inverse Park Transform/1
  Vd/1 -> Mux/1
  Inverse Park Transform/1 -> Vabc/1
  Vq/1 -> Mux/2

== system single_motor_fix/Controller1/FOC/thm2the ==
  thm : Inport
  Constant : Constant  Value=2*pi
  Mod : Math  Operator=mod  SignedPower=on
  PolePairs : Gain  Gain=p
  the : Outport  VectorParamsAs1DForOutWhenUnconnected=off
  wires:
  Constant/1 -> Mod/2
  PolePairs/1 -> Mod/1
  Mod/1 -> the/1
  thm/1 -> PolePairs/1

== system single_motor_fix/Controller1/FOC/wm2we ==
  wm : Inport
  PolePairs : Gain  Gain=p
  we : Outport  VectorParamsAs1DForOutWhenUnconnected=off
  wires:
  wm/1 -> PolePairs/1
  PolePairs/1 -> we/1

== matlab function single_motor_fix/Controller1/FOC/CurrentController/MATLAB Function ==
  data: z_q input; Vq output; i_q_ref input; i_q input; i_d input; we input; Vd output; dz_q output; e_q_bar output; Rs parameter; Ld parameter; Lq parameter; Phi parameter
function [Vq, Vd, dz_q, e_q_bar] = smc_ctrl(z_q, i_q_ref, i_q, i_d, we, Rs, Ld, Lq, Phi)
%#codegen
% ============================================================
%  PMSM 超螺旋滑模电流控制器
%  Rs, Ld, Lq, Phi, p 及滑模增益均由 Parameter 作用域提供
% ============================================================

%% ---------- 滑模参数 (仍然写死, 因为它们只属于控制器) ----------
r1  = 0.5;   r2  = 1.5;
rho1 = 0.5;  rho2 = 1.5;

k_q1 = -5000;  k_q2 = -4000;
k_d1 = -5000;  k_d2 = -4000;

lam_q1 = 50;   lam_q2 = 50;

%% ---------- 滑模面 ----------
e_q_bar = i_q - z_q;

%% ---------- 迭代部分的导数 (积分交给 Simulink) ----------
e_z  = z_q - i_q_ref;
dz_q = -lam_q1 * sig(e_z, rho1) - lam_q2 * sig(e_z, rho2);

%% ---------- u_q (非迭代) ----------
Vq = Lq * ( dz_q ...
             + k_q1 * sig(e_q_bar, r1) ...
             + k_q2 * sig(e_q_bar, r2) ) ...
      + Rs * z_q ...
      + Ld * we * i_d ...
      + we * Phi ;

%% ---------- u_d (非迭代) ----------
Vd = Ld * ( k_d1 * sig(i_d, r1) ...
             + k_d2 * sig(i_d, r2) ) ...
      + Rs * i_d ...
      + Lq * we * i_q;

end

function y = sig(x, r)
    y = abs(x)^r * sign(x);
end

== matlab function single_motor_fix/MATLAB Function ==
  data: theta_ref input; omega_cmd output; dalpha output; e input; alpha_bar input
function [omega_cmd, dalpha] = ft_dsc_ctrl(theta_ref, e, alpha_bar)
%#codegen
% 固定时间动态面 + 固定时间控制器
% 本块只算导数 dalpha 与控制量；alpha_bar 由外部 Integrator 积分

% ---------- 固定时间动态面参数 ----------
tau  = 0.005;
kf1  = 30;   pf1 = 0.5;
kf2  = 15;   pf2 = 1.5;

% ---------- 控制器参数 ----------
k1 = 5;  p1 = 0.5;
k2 =  5;  p2 = 1.5;

sig = @(v,p) (abs(v)^p) * sign(v);

% ---------- 动态面滤波器：只输出导数 ----------
delta  = alpha_bar - theta_ref;
dalpha = -( kf1*sig(delta,pf1) + kf2*sig(delta,pf2) ) / tau;

% ---------- om_ref 的估计 = alpha_bar 的导数 ----------
om_ref_hat = dalpha;

% ---------- 控制律 ----------
u = om_ref_hat + k1*sig(e,p1) + k2*sig(e,p2);

% ---------- ±50 饱和 ----------
omega_cmd = min(max(u, -50), 50);

end

== matlab function single_motor_fix/Controller1/FOC/VelocityController/MATLAB Function ==
  data: w_ref input; u_cmd output; w_m input; bar_w input; xi input; Jm parameter; Dm parameter; dot_bar_w output; dot_xi output
function [u_cmd, dot_bar_w, dot_xi] = FixedTimeController(w_ref, w_m, bar_w, xi, Jm, Dm)

    lambda1  = 5;   lambda2 = 5;   lambda3 = 6;
    tau      = 0.5; vartheta = 1.5;
    k_w = 6; k1 = 5; k2 = 5;

    k_i = 20;

    kappa0 = 30;     % 线性积分增益（新增，压制小误差）
    kappa1 = 20;     % 固定时间项增益
    kappa2 = 20;
    alpha1 = 0.5;
    alpha2 = 1.5;

    pow_func = @(x, gamma) abs(x)^gamma * sign(x);

    % 公式(117) 滤波器
    e_w = bar_w - w_ref;
    dot_bar_w = (1/tau) * ( -lambda1 * pow_func(e_w, 0.5) ...
                            -lambda2 * pow_func(e_w, vartheta) ...
                            -lambda3 * e_w );

    s   = w_m - bar_w;
    e_v = w_m - w_ref;

    % 混合固定时间积分
    dot_xi = kappa0 * e_v ...
           + kappa1 * pow_func(e_v, alpha1) ...
           + kappa2 * pow_func(e_v, alpha2);

    TL_hat_int = k_i * xi;

    feedback = -k_w * s ...
               - k1 * pow_func(s, 0.5) ...
               - k2 * pow_func(s, vartheta);

    u_cmd = Jm * dot_bar_w + Dm * bar_w - TL_hat_int + feedback;
end

== matlab function single_motor_fix/Controller/FOC/CurrentController/MATLAB Function ==
  data: z_q input; Vq output; i_q_ref input; i_q input; i_d input; we input; Vd output; dz_q output; e_q_bar output; Rs parameter; Ld parameter; Lq parameter; Phi parameter
function [Vq, Vd, dz_q, e_q_bar] = smc_ctrl(z_q, i_q_ref, i_q, i_d, we, Rs, Ld, Lq, Phi)
%#codegen
% ============================================================
%  PMSM 超螺旋滑模电流控制器
%  Rs, Ld, Lq, Phi, p 及滑模增益均由 Parameter 作用域提供
% ============================================================

%% ---------- 滑模参数 (仍然写死, 因为它们只属于控制器) ----------
r1  = 0.5;   r2  = 1.5;
rho1 = 0.5;  rho2 = 1.5;

k_q1 = -5000;  k_q2 = -4000;
k_d1 = -5000;  k_d2 = -4000;

lam_q1 = 50;   lam_q2 = 50;

%% ---------- 滑模面 ----------
e_q_bar = i_q - z_q;

%% ---------- 迭代部分的导数 (积分交给 Simulink) ----------
e_z  = z_q - i_q_ref;
dz_q = -lam_q1 * sig(e_z, rho1) - lam_q2 * sig(e_z, rho2);

%% ---------- u_q (非迭代) ----------
Vq = Lq * ( dz_q ...
             + k_q1 * sig(e_q_bar, r1) ...
             + k_q2 * sig(e_q_bar, r2) ) ...
      + Rs * z_q ...
      + Ld * we * i_d ...
      + we * Phi ;

%% ---------- u_d (非迭代) ----------
Vd = Ld * ( k_d1 * sig(i_d, r1) ...
             + k_d2 * sig(i_d, r2) ) ...
      + Rs * i_d ...
      + Lq * we * i_q;

end

function y = sig(x, r)
    y = abs(x)^r * sign(x);
end
